simulink model "balance_and_leg_control"  (R2021b)
settings: Solver=ode4  StartTime=0.0  StopTime=12  FixedStep=1e-4  RelTol=1e-3
undefined symbols (not defined in the file): balance_controller_t, body, leg1, leg2, leg_controller_t, leg_fit_t, leg_t, param_t, sigbuilder_block, wheel, X, Y, Z
libraries: sm_lib x59, nesl_utility x15, slpidlib x2
(part 1 of 2)
settings Model: SimulationMode=accelerator  Creator=thinkpad  LastModifiedBy=thinkpad
settings OptimizationCC: DefaultUnderspecifiedDataType=single
settings ExplorerConfigSet: InternalSimMechanicsExplorerSettings="<ExplorerConfiguration><canonicalview>default</canonicalview><AnimationSetting><BasePlaybackSpeed>1.0</BasePlaybackSpeed><PlaybackSpeedFactor>1.0</PlaybackSpeedFactor></AnimationSetting><TilePanel><TileInfo><Tiles Columns=\"1\" Count=\"1\" Rows=\"1\"><Column Weight=\"1\"/><Row Weight=\"1\"/><Tile Height=\"1\" Width=\"1\" X=\"0\" Y=\"0\"/></Tiles></TileInfo><SceneInfo><SceneViewer><BGColor><R>0.815686285495758057</R><G>0.815686285495758057</G><B>0.815686285495758057</B></BGColor><Camera><DoPerspective>off</DoPerspective><Position><X>0.307352454887792503</X><Y>-1.00000000399907174</Y><Z>0.174322899702416489</Z></Position><Center><X>0.307352454887792503</X><Y>-3.99907176817926313e-09</Y><Z>0.174322899702416489</Z></Center><Up><X>0</X><Y>-0</Y><Z>1</Z></Up><ViewLimDist>1</ViewLimDist><YLim>0.280830658411598988</YLim><XLim>0.503375708473620787</XLim></Camera></SceneViewer></SceneInfo></TilePanel><MechEditorPanel><Cameras/><GfxPanelCameraMap/><VideoCreator><PlaybackSpeedRatio>1.0</PlaybackSpeedRatio><FrameRate>30</FrameRate><VideoFormat>Motion JPEG AVI</VideoFormat><FrameSize>[800 600]</FrameSize></VideoCreator></MechEditorPanel></ExplorerConfiguration>"

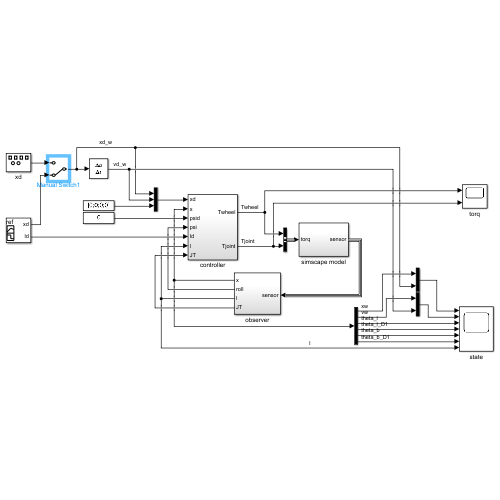
[thumbnail: Simulink's stored preview of the top-level diagram]
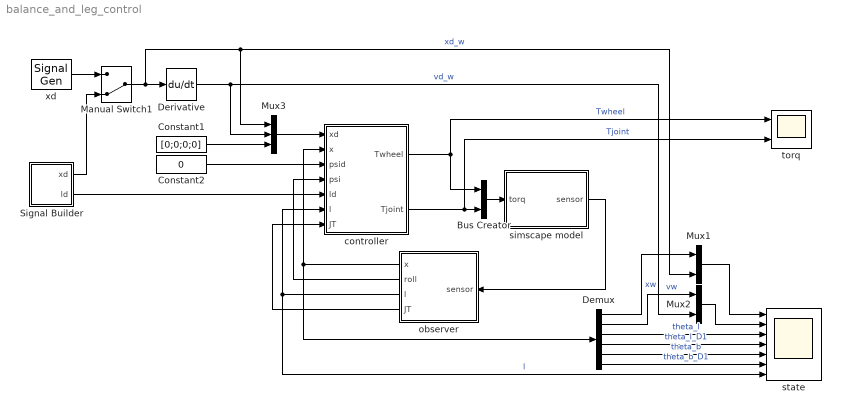
== system balance_and_leg_control ==
  Bus Creator : BusCreator  Inputs=2
  Constant1 : Constant  Value=[0;0;0;0]
  Constant2 : Constant  Value=0
  Demux : Demux  Outputs=6
  Derivative : Derivative
  Manual Switch1 : ManualSwitch  CurrentSetting=0
  Mux1 : Mux  Inputs=2
  Mux2 : Mux  Inputs=2
  Mux3 : Mux  Inputs=3
  Signal Builder : Subsystem  Tag=STV Subsys  LoadFcn=sigbuilder_block('load');  StartFcn=sigbuilder_block('start');  StopFcn=sigbuilder_block('stop');  ClipboardFcn=sigbuilder_block('clipboard');  mask(Sigbuilder block){tuvar=[0:10]}
      mask help: Simulink:masks:SigbuilderBlock_MD
      mask init:
      | if ~strcmp(get_param(bdroot(gcbh),'SimulationStatus'),'stopped') tuvar = sigbuilder_block('maskInit'); end
      settings: CopyFcn=sigbuilder_block('copy');  DeleteFcn=sigbuilder_block('delete');  ModelCloseFcn=sigbuilder_block('modelClose');  PreSaveFcn=sigbuilder_block('preSave');  PauseFcn=sigbuilder_block('pause');  ContinueFcn=sigbuilder_block('continue');  NameChangeFcn=sigbuilder_block('namechange');  OpenFcn=sigbuilder_block('open',[427.2 154.8 550.8 400.2 ]);  CloseFcn=sigbuilder_block('close');
      mask Display: plot(0, 0, 100, 100,[2, 2, 32, 32, 2], [68, 8, 8, 68, 68],[32, 2], [38, 38], [32, 19, 2],[53, 60, 44], [32, 17, 17, 2],[16, 16, 31, 31]);txt = getActiveGroup(gcbh);text(2, 100, txt,'verticalAlignment', 'top');
  controller : Subsystem
  observer : Subsystem
  simscape model : Subsystem
  state : Scope  NumInputPorts=7
  torq : Scope  NumInputPorts=2
  xd : SignalGenerator  WaveForm=square  Amplitude=0  Frequency=0.1
  wires:
  Manual Switch1/1 -> Mux1/2, Mux3/1, Derivative/1  "xd_w"
  Mux3/1 -> controller/1(xd)
  Constant1/1 -> Mux3/3
  Derivative/1 -> Mux3/2, Mux2/2  "vd_w"
  xd/1 -> Manual Switch1/1
  Signal Builder/1(xd) -> Manual Switch1/2
  controller/1(Twheel) -> torq/1, Bus Creator/1  "Twheel"
  controller/2(Tjoint) -> torq/2, Bus Creator/2  "Tjoint"
  Signal Builder/2(ld) -> controller/5(ld)
  Bus Creator/1 -> simscape model/1(torq)
  observer/4(JT) -> controller/7(JT)
  observer/3(l) -> state/7, controller/6(l)  "l"
  observer/2(roll) -> controller/4(psi)
  observer/1(x) -> controller/2(x), Demux/1
  Constant2/1 -> controller/3(psid)
  simscape model/1(sensor) -> observer/1(sensor)
  Demux/1 -> Mux1/1  "xw"
  Demux/2 -> Mux2/1  "vw"
  Mux1/1 -> state/1
  Mux2/1 -> state/2
  Demux/3 -> state/3  "theta_l"
  Demux/6 -> state/6  "theta_b_D1"
  Demux/5 -> state/5  "theta_b"
  Demux/4 -> state/4  "theta_l_D1"

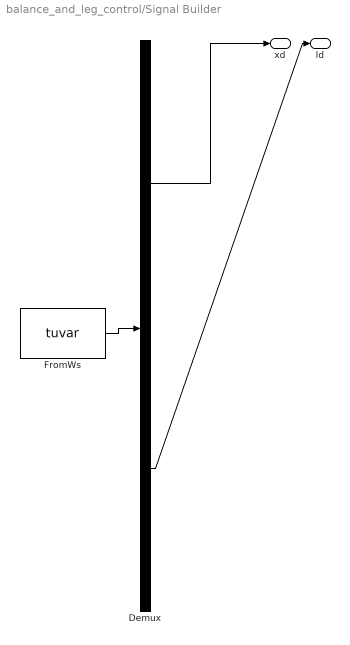
== system balance_and_leg_control/Signal Builder ==
  Demux : Demux  Tag=STV Demux  Outputs=2
      settings: DisplayOption=none
  FromWs : FromWorkspace  Tag=STV FromWs  VariableName=tuvar
      SigBuilderData=|
      | common.afterFinalStr = 'Extrapolate'
      | common.sampleTime = 0
      | dataSet.timeRange = [0 20]
      | dataSet.name = 'ref'
      | sbobj.Groups.Name = 'ref'
      | sbobj.Groups.Signals(1).Name = 'xd'
      | sbobj.Groups.Signals(1).XData = [0 1.5 2 4.5 7 10 20]
      | sbobj.Groups.Signals(1).YData = [0.1 -3.5 -3.5 4 4 0 0]
      | sbobj.Groups.Signals(2).Name = 'ld'
      | sbobj.Groups.Signals(2).XData = [0 20]
      | sbobj.Groups.Signals(2).YData = [0.24 0.24]
      | sbobj.Groups.TimeRange = [0 20]
  xd : Outport  Tag=STV Outport
  ld : Outport  Tag=STV Outport  Port=2
  wires:
  Demux/1 -> xd/1
  FromWs/1 -> Demux/1
  Demux/2 -> ld/1

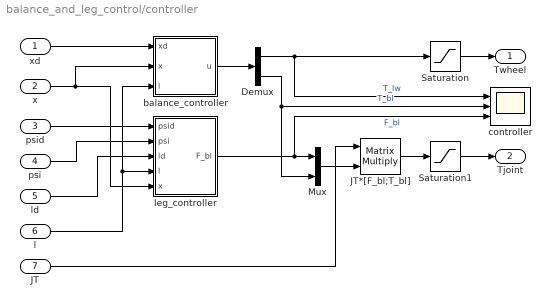
== system balance_and_leg_control/controller ==
  xd : Inport
  x : Inport  Port=2
  psid : Inport  Port=3
  psi : Inport  Port=4
  ld : Inport  Port=5
  l : Inport  Port=6
  JT : Inport  Port=7
  Demux : Demux  Outputs=2
  JT*[F_bl;T_bl] : Product  Multiplication=Matrix(*)
  Mux : Mux  Inputs=2
  Saturation : Saturate  UpperLimit=8  LowerLimit=-8
  Saturation1 : Saturate  UpperLimit=[70 70]  LowerLimit=-[70 70]
  balance_controller : Subsystem
  controller : Scope  NumInputPorts=3
  leg_controller : Subsystem
  Twheel : Outport
  Tjoint : Outport  Port=2
  wires:
  xd/1 -> balance_controller/1(xd)
  x/1 -> leg_controller/5(x), balance_controller/2(x)
  balance_controller/1(u) -> Demux/1
  Demux/1 -> Saturation/1, controller/1  "T_lw"
  leg_controller/1(F_bl) -> controller/3, Mux/1  "F_bl"
  Demux/2 -> controller/2, Mux/2  "T_bl"
  l/1 -> balance_controller/3(l), leg_controller/4(l)
  psid/1 -> leg_controller/1(psid)
  psi/1 -> leg_controller/2(psi)
  ld/1 -> leg_controller/3(ld)
  Mux/1 -> JT*[F_bl;T_bl]/2
  JT*[F_bl;T_bl]/1 -> Saturation1/1
  JT/1 -> JT*[F_bl;T_bl]/1
  Saturation/1 -> Twheel/1
  Saturation1/1 -> Tjoint/1

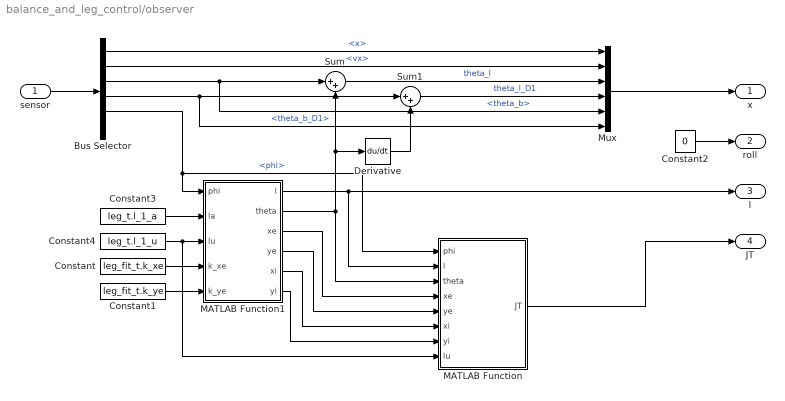
== system balance_and_leg_control/observer ==
  sensor : Inport
  Bus Selector : BusSelector  OutputSignals=x,vx,theta_b,theta_b_D1,phi,phi_D1
  Constant : Constant  Value=leg_fit_t.k_xe
  Constant1 : Constant  Value=leg_fit_t.k_ye
  Constant2 : Constant  Value=0
  Constant3 : Constant  Value=leg_t.l_1_a
  Constant4 : Constant  Value=leg_t.l_1_u
  Derivative : Derivative
  MATLAB Function : MATLAB Function  TreatAsAtomicUnit=on
  MATLAB Function1 : MATLAB Function  TreatAsAtomicUnit=on
  Mux : Mux  Inputs=6
  Sum : Sum  Inputs=|++
  Sum1 : Sum  Inputs=|++
  x : Outport
  roll : Outport  Port=2
  l : Outport  Port=3
  JT : Outport  Port=4
  wires:
  MATLAB Function1/1(l) -> l/1, MATLAB Function/2(l)
  MATLAB Function1/2(theta) -> Sum/2, Derivative/1, MATLAB Function/3(theta)
  MATLAB Function/1(JT) -> JT/1
  sensor/1 -> Bus Selector/1
  Mux/1 -> x/1
  Bus Selector/1 -> Mux/1  "<x>"
  Bus Selector/2 -> Mux/2  "<vx>"
  Constant2/1 -> roll/1
  Bus Selector/3 -> Sum/1, Mux/5  "<theta_b>"
  Bus Selector/4 -> Sum1/1, Mux/6  "<theta_b_D1>"
  Bus Selector/5 -> MATLAB Function1/1(phi), MATLAB Function/1(phi)  "<phi>"
  Constant/1 -> MATLAB Function1/4(k_xe)
  Constant1/1 -> MATLAB Function1/5(k_ye)
  Sum/1 -> Mux/3  "theta_l"
  Sum1/1 -> Mux/4  "theta_l_D1"
  Derivative/1 -> Sum1/2
  Constant3/1 -> MATLAB Function1/2(la)
  Constant4/1 -> MATLAB Function1/3(lu), MATLAB Function/8(lu)
  MATLAB Function1/3(xe) -> MATLAB Function/4(xe)
  MATLAB Function1/4(ye) -> MATLAB Function/5(ye)
  MATLAB Function1/5(xi) -> MATLAB Function/6(xi)
  MATLAB Function1/6(yi) -> MATLAB Function/7(yi)

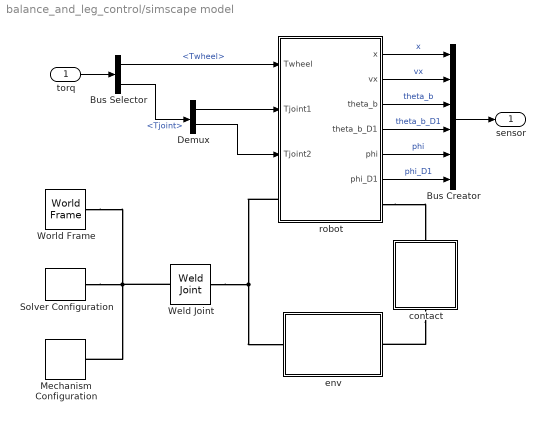
== system balance_and_leg_control/simscape model ==
  torq : Inport
  Bus Creator : BusCreator  Inputs=6
  Bus Selector : BusSelector  OutputSignals=Twheel,Tjoint
  Demux : Demux  Outputs=2
  Mechanism Configuration : sm_lib/Utilities/Mechanism Configuration  UniformGravity=Constant  GravityVector=[0 0 -9.81]  GravityUnits=m/s^2  LinearizationDelta=0.001  JointModeTransitionNonlinearIterations=2
  Solver Configuration : nesl_utility/Solver Configuration  PhysicalDomain=network_engine_domain  SubClassName=solver  LeftPortType=input  RightPortType=generic  Tones=[]  Harmonics=[]  SimulateNoise=off  Profile=off  UseLocalSampling=off  EnableSwitchedLinearOptims=on  FrequencyDomain=off  UseCCode=off  RelTol=0.001  AbsTol=1e-06  MinStep=1e-09  ToWorkspace=off  RevertToSquareIcSolve=off  NumHomotopyIterations=100  PhasorMode=off  PhasorModeNumHarmonics=1  DoDC=off  ResidualTolerance=1e-09  UseLocalSolver=off  LocalSolverChoice=NE_BACKWARD_EULER_ADVANCER  LocalSolverSampleTime=0.001  DoFixedCost=off  MaxNonlinIter=3  MaxModeIter=2  ComputeImpulses=off  ImpulseIterations=2  LinearAlgebra=Sparse  EquationFormulation=NE_TIME_EF  DelaysMemoryBudget=1024  AutomaticFiltering=on  FilteringTimeConstant=0.001  PartitionStorageMethod=AS_NEEDED  PartitionMemoryBudget=1024  PartitionMethod=FAST
      settings: SourceProductBaseCode=PW,SS
  Weld Joint : sm_lib/Joints/Weld Joint  JointMode=Normal  SenseConstraintForce=off  SenseConstraintForceX=off  SenseConstraintForceY=off  SenseConstraintForceZ=off  SenseConstraintTorque=off  SenseConstraintTorqueX=off  SenseConstraintTorqueY=off  SenseConstraintTorqueZ=off  SenseTotalForce=off  SenseTotalForceX=off  SenseTotalForceY=off  SenseTotalForceZ=off  SenseTotalTorque=off  SenseTotalTorqueX=off  SenseTotalTorqueY=off  SenseTotalTorqueZ=off  CompositeWrenchDir=FollowerOnBase  CompositeWrenchFrame=BaseFrame
  World Frame : sm_lib/Frames and Transforms/World Frame
  contact : Subsystem
      settings: PortSchema="{\"entries\":[{\"content\":{\"sides\":[{\"content\":{\"connectorIds\":[]},\"type\":\"ConnectorPlacement.EquallySpacedRectSide\",\"uuid\":\"948d884d-a2bb-4982-bec2-8891ab05edb1\"},{\"content\":{\"connectorIds\":[],\"side\":\"RIGHT\"},\"type\":\"ConnectorPlacement.EquallySpacedRectSide\",\"uuid\":\"1ab48329-b8c1-41fb-bc52-c8a32a07fc10\"},{\"content\":{\"connectorIds\":[\"LConn1\"],\"side\":\"TOP\"},\"type\":\"ConnectorPlacement.EquallySpacedRectSide\",\"uuid\":\"2430d379-17bc-45a7-9277-8300fd306697\"},{\"content\":{\"connectorIds\":[\"RConn1\"],\"side\":\"BOTTOM\"},\"type\":\"ConnectorPlacement.EquallySpacedRectSide\",\"uuid\":\"c2c22df6-47ef-4364-9ed6-2fe5d2ebd561\"}]},\"type\":\"ConnectorPlacement.EquallySpacedConnector\",\"uuid\":\"bd96c317-3050-474a-affa-ffce42783eb1\"}],\"packageUris\":[\"http://schema.mathworks.com/mf0/Connector/R2020b\"],\"version\":\"1.0\"}"
  env : Subsystem
  robot : Subsystem
  sensor : Outport
  wires:
  torq/1 -> Bus Selector/1
  Bus Selector/2 -> Demux/1  "<Tjoint>"
  Demux/1 -> robot/2(Tjoint1)
  Demux/2 -> robot/3(Tjoint2)
  Bus Creator/1 -> sensor/1
  robot/1(x) -> Bus Creator/1  "x"
  robot/2(vx) -> Bus Creator/2  "vx"
  robot/3(theta_b) -> Bus Creator/3  "theta_b"
  robot/4(theta_b_D1) -> Bus Creator/4  "theta_b_D1"
  robot/5(phi) -> Bus Creator/5  "phi"
  robot/6(phi_D1) -> Bus Creator/6  "phi_D1"
  Bus Selector/1 -> robot/1(Twheel)  "<Twheel>"
  connections:
  World Frame/RConn1 -- Weld Joint/LConn1 -- Mechanism Configuration/RConn1 -- Solver Configuration/RConn1
  contact/RConn1 -- env/RConn1
  Weld Joint/RConn1 -- env/LConn1 -- robot/LConn1
  robot/RConn1 -- contact/LConn1

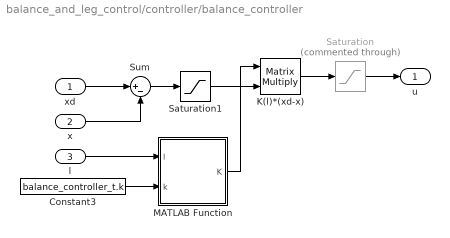
== system balance_and_leg_control/controller/balance_controller ==
  xd : Inport
  x : Inport  Port=2
  l : Inport  Port=3
  Constant3 : Constant  Value=balance_controller_t.k
  K(l)*(xd-x) : Product  Multiplication=Matrix(*)
  MATLAB Function : MATLAB Function  TreatAsAtomicUnit=on
  Saturation : Saturate  Commented=through  UpperLimit=1  LowerLimit=-1
  Saturation1 : Saturate  UpperLimit=[0.5,3,inf,inf,inf,inf]  LowerLimit=-[0.5,3,inf,inf,inf,inf]
  Sum : Sum  Inputs=|+-
  u : Outport
  wires:
  Saturation/1 -> u/1
  Saturation1/1 -> K(l)*(xd-x)/2
  MATLAB Function/1(K) -> K(l)*(xd-x)/1
  l/1 -> MATLAB Function/1(l)
  x/1 -> Sum/2
  xd/1 -> Sum/1
  Sum/1 -> Saturation1/1
  K(l)*(xd-x)/1 -> Saturation/1
  Constant3/1 -> MATLAB Function/2(k)

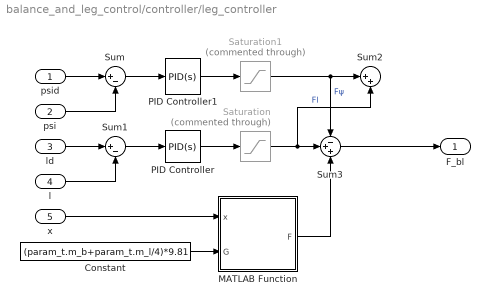
== system balance_and_leg_control/controller/leg_controller ==
  psid : Inport
  psi : Inport  Port=2
  ld : Inport  Port=3
  l : Inport  Port=4
  x : Inport  Port=5
  Constant : Constant  Value=(param_t.m_b+param_t.m_l/4)*9.81
  MATLAB Function : MATLAB Function  TreatAsAtomicUnit=on
  PID Controller : slpidlib/PID Controller  Controller=PID  Form=Parallel  TimeDomain=Continuous-time  UseExternalTs=off  SampleTime=-1  IntegratorMethod=Forward Euler  FilterMethod=Forward Euler  ControllerParametersSource=internal  P=leg_controller_t.l.kp  I=leg_controller_t.l.ki  D=leg_controller_t.l.kd  UseFilter=on  N=100  TunerSelectOption=Transfer Function Based (PID Tuner App)  InitialConditionSource=internal  InitialConditionForIntegrator=0  InitialConditionForFilter=0  DifferentiatorICPrevScaledInput=0  ExternalReset=none  TrackingMode=off  Kt=1  LimitOutput=off  SatLimitsSource=internal  UpperSaturationLimit=inf  LowerSaturationLimit=-inf  LinearizeAsGain=on  AntiWindupMode=none  Kb=1  POutMin=[]  POutMax=[]  IOutMin=[]  IOutMax=[]  DOutMin=[]  DOutMax=[]  NOutMin=[]  NOutMax=[]  SumOutMin=[]  SumOutMax=[]  SaturationOutMin=[]  SaturationOutMax=[]  PParamMin=[]  PParamMax=[]  IParamMin=[]  IParamMax=[]  DParamMin=[]  DParamMax=[]  NParamMin=[]  NParamMax=[]  KbParamMin=[]  KbParamMax=[]  KtParamMin=[]  KtParamMax=[]  KbOutMin=[]  KbOutMax=[]  KtOutMin=[]  KtOutMax=[]  IntegratorOutMin=[]  IntegratorOutMax=[]  FilterOutMin=[]  FilterOutMax=[]  SumI1OutMin=[]  SumI1OutMax=[]  SumI2OutMin=[]  SumI2OutMax=[]  SumI3OutMin=[]  SumI3OutMax=[]  SumI4OutMin=[]  SumI4OutMax=[]  SumDOutMin=[]  SumDOutMax=[]  DifferentiatorOutMin=[]  DifferentiatorOutMax=[]  FilterDiffOutCoefMin=[]  FilterDiffOutCoefMax=[]  ReciprocalOutMin=[]  ReciprocalOutMax=[]  SumDenOutMin=[]  SumDenOutMax=[]  SumNumOutMin=[]  SumNumOutMax=[]  DivideOutMin=[]  DivideOutMax=[]  UdiffTsProdOutMin=[]  UdiffTsProdOutMax=[]  NTsProdOutMin=[]  NTsProdOutMax=[]  UintegralTsProdOutMin=[]  UintegralTsProdOutMax=[]  UngainTsProdOutMin=[]  UngainTsProdOutMax=[]  IntegratorContinuousStateAttributes=''  IntegratorStateMustResolveToSignalObject=off  IntegratorRTWStateStorageClass=Auto  FilterContinuousStateAttributes=''  FilterStateMustResolveToSignalObject=off  FilterRTWStateStorageClass=Auto  ParallelPVariant=InternalParameters  IdealPVariant=Disabled  IVariant=InternalParameters  DVariant=InternalParameters  IntegratorVariant=Continuous  SatVariant=Disabled  AWVariant=Passthrough  PCopyVariant=Disabled  TRVariant=Disabled  FdbkBlocksVariant=Forward  IdealPFdbkVariant=Disabled  SatFdbkVariant=Disabled  DerivativeFilterVariant=ContFilter  NVariant=InternalParameters  NCopyVariant=Disabled  FilterICVariant=InternalICsFilter  IntegratorICVariant=InternalICs  ExternalResetVariant=Disabled  TRSumVariant=Passthrough  SumFdbkVariant=Disabled  SumVariant=Sum_PID  TsampFilterVariant=InternalTs  TsampNgainVariant=Passthrough  TsampIntegralVariant=Passthrough  ExternalSaturationOutDataTypeStr=Inherit: Same as second input
  PID Controller1 : slpidlib/PID Controller  Controller=PID  Form=Parallel  TimeDomain=Continuous-time  UseExternalTs=off  SampleTime=-1  IntegratorMethod=Forward Euler  FilterMethod=Forward Euler  ControllerParametersSource=internal  P=leg_controller_t.psi.kp  I=leg_controller_t.psi.ki  D=leg_controller_t.psi.kd  UseFilter=on  N=100  TunerSelectOption=Transfer Function Based (PID Tuner App)  InitialConditionSource=internal  InitialConditionForIntegrator=0  InitialConditionForFilter=0  DifferentiatorICPrevScaledInput=0  ExternalReset=none  TrackingMode=off  Kt=1  LimitOutput=off  SatLimitsSource=internal  UpperSaturationLimit=inf  LowerSaturationLimit=-inf  LinearizeAsGain=on  AntiWindupMode=none  Kb=1  POutMin=[]  POutMax=[]  IOutMin=[]  IOutMax=[]  DOutMin=[]  DOutMax=[]  NOutMin=[]  NOutMax=[]  SumOutMin=[]  SumOutMax=[]  SaturationOutMin=[]  SaturationOutMax=[]  PParamMin=[]  PParamMax=[]  IParamMin=[]  IParamMax=[]  DParamMin=[]  DParamMax=[]  NParamMin=[]  NParamMax=[]  KbParamMin=[]  KbParamMax=[]  KtParamMin=[]  KtParamMax=[]  KbOutMin=[]  KbOutMax=[]  KtOutMin=[]  KtOutMax=[]  IntegratorOutMin=[]  IntegratorOutMax=[]  FilterOutMin=[]  FilterOutMax=[]  SumI1OutMin=[]  SumI1OutMax=[]  SumI2OutMin=[]  SumI2OutMax=[]  SumI3OutMin=[]  SumI3OutMax=[]  SumI4OutMin=[]  SumI4OutMax=[]  SumDOutMin=[]  SumDOutMax=[]  DifferentiatorOutMin=[]  DifferentiatorOutMax=[]  FilterDiffOutCoefMin=[]  FilterDiffOutCoefMax=[]  ReciprocalOutMin=[]  ReciprocalOutMax=[]  SumDenOutMin=[]  SumDenOutMax=[]  SumNumOutMin=[]  SumNumOutMax=[]  DivideOutMin=[]  DivideOutMax=[]  UdiffTsProdOutMin=[]  UdiffTsProdOutMax=[]  NTsProdOutMin=[]  NTsProdOutMax=[]  UintegralTsProdOutMin=[]  UintegralTsProdOutMax=[]  UngainTsProdOutMin=[]  UngainTsProdOutMax=[]  IntegratorContinuousStateAttributes=''  IntegratorStateMustResolveToSignalObject=off  IntegratorRTWStateStorageClass=Auto  FilterContinuousStateAttributes=''  FilterStateMustResolveToSignalObject=off  FilterRTWStateStorageClass=Auto  ParallelPVariant=InternalParameters  IdealPVariant=Disabled  IVariant=InternalParameters  DVariant=InternalParameters  IntegratorVariant=Continuous  SatVariant=Disabled  AWVariant=Passthrough  PCopyVariant=Disabled  TRVariant=Disabled  FdbkBlocksVariant=Forward  IdealPFdbkVariant=Disabled  SatFdbkVariant=Disabled  DerivativeFilterVariant=ContFilter  NVariant=InternalParameters  NCopyVariant=Disabled  FilterICVariant=InternalICsFilter  IntegratorICVariant=InternalICs  ExternalResetVariant=Disabled  TRSumVariant=Passthrough  SumFdbkVariant=Disabled  SumVariant=Sum_PID  TsampFilterVariant=InternalTs  TsampNgainVariant=Passthrough  TsampIntegralVariant=Passthrough  ExternalSaturationOutDataTypeStr=Inherit: Same as second input
  Saturation : Saturate  Commented=through  UpperLimit=30  LowerLimit=-30
  Saturation1 : Saturate  Commented=through  UpperLimit=30  LowerLimit=-30
  Sum : Sum  Inputs=|+-
  Sum1 : Sum  Inputs=|+-
  Sum2 : Sum  Inputs=|++
  Sum3 : Sum  Inputs=-++
  F_bl : Outport
  wires:
  psi/1 -> Sum/2
  l/1 -> Sum1/2
  ld/1 -> Sum1/1
  psid/1 -> Sum/1
  Sum1/1 -> PID Controller/1
  Sum/1 -> PID Controller1/1
  PID Controller1/1 -> Saturation1/1
  PID Controller/1 -> Saturation/1
  Saturation1/1 -> Sum3/1, Sum2/1  "Fψ"
  Saturation/1 -> Sum2/2, Sum3/2  "Fl"
  Sum3/1 -> F_bl/1
  Constant/1 -> MATLAB Function/2(G)
  x/1 -> MATLAB Function/1(x)
  MATLAB Function/1(F) -> Sum3/3

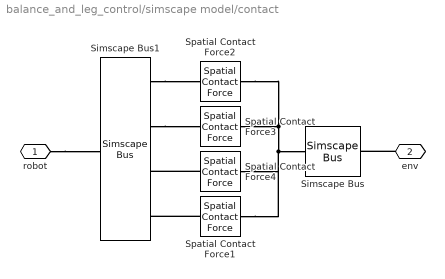
== system balance_and_leg_control/simscape model/contact ==
  Simscape Bus : SimscapeBus  HierarchyStrings=ground
  Simscape Bus1 : SimscapeBus  HierarchyStrings=body;leg1;leg2;wheel
  Spatial Contact Force1 : sm_lib/Forces and Torques/Spatial Contact Force  CoefficientOfDynamicFriction=0.3  CoefficientOfStaticFriction=0.5  SenseContactBaseRotation=off  SenseContactBaseTranslation=off  NormalDamping=1e5  NormalDampingUnits=N/(m/s)  SenseContactFollowerRotation=off  SenseContactFollowerTranslation=off  SenseContactSignal=off  NormalStiffness=1e6  NormalStiffnessUnits=N/m  FrictionalCriticalVelocity=1e-3  FrictionalCriticalVelocityUnits=m/s  ZeroCrossDetectContactStartAndEnd=off  FrictionType=SmoothStickSlip  SenseFrictionalForceMagnitude=off  SenseNormalForceMagnitude=off  NormalForceType=SmoothSpringDamper  SenseNormalVelocity=off  SenseSeparationDistance=off  SenseTangentialVelocity=off  SenseTangentialVelocityMagnitude=off  NormalTransitionRegionWidth=1e-4  NormalTransitionRegionWidthUnits=m
  Spatial Contact Force2 : sm_lib/Forces and Torques/Spatial Contact Force  CoefficientOfDynamicFriction=0.3  CoefficientOfStaticFriction=0  SenseContactBaseRotation=off  SenseContactBaseTranslation=off  NormalDamping=1e5  NormalDampingUnits=N/(m/s)  SenseContactFollowerRotation=off  SenseContactFollowerTranslation=off  SenseContactSignal=off  NormalStiffness=1e6  NormalStiffnessUnits=N/m  FrictionalCriticalVelocity=1e-3  FrictionalCriticalVelocityUnits=m/s  ZeroCrossDetectContactStartAndEnd=off  FrictionType=SmoothStickSlip  SenseFrictionalForceMagnitude=off  SenseNormalForceMagnitude=off  NormalForceType=SmoothSpringDamper  SenseNormalVelocity=off  SenseSeparationDistance=off  SenseTangentialVelocity=off  SenseTangentialVelocityMagnitude=off  NormalTransitionRegionWidth=1e-4  NormalTransitionRegionWidthUnits=m
  Spatial Contact Force3 : sm_lib/Forces and Torques/Spatial Contact Force  CoefficientOfDynamicFriction=0.3  CoefficientOfStaticFriction=0  SenseContactBaseRotation=off  SenseContactBaseTranslation=off  NormalDamping=1e5  NormalDampingUnits=N/(m/s)  SenseContactFollowerRotation=off  SenseContactFollowerTranslation=off  SenseContactSignal=off  NormalStiffness=1e6  NormalStiffnessUnits=N/m  FrictionalCriticalVelocity=1e-3  FrictionalCriticalVelocityUnits=m/s  ZeroCrossDetectContactStartAndEnd=off  FrictionType=SmoothStickSlip  SenseFrictionalForceMagnitude=off  SenseNormalForceMagnitude=off  NormalForceType=SmoothSpringDamper  SenseNormalVelocity=off  SenseSeparationDistance=off  SenseTangentialVelocity=off  SenseTangentialVelocityMagnitude=off  NormalTransitionRegionWidth=1e-4  NormalTransitionRegionWidthUnits=m
  Spatial Contact Force4 : sm_lib/Forces and Torques/Spatial Contact Force  CoefficientOfDynamicFriction=0.3  CoefficientOfStaticFriction=0  SenseContactBaseRotation=off  SenseContactBaseTranslation=off  NormalDamping=1e5  NormalDampingUnits=N/(m/s)  SenseContactFollowerRotation=off  SenseContactFollowerTranslation=off  SenseContactSignal=off  NormalStiffness=1e6  NormalStiffnessUnits=N/m  FrictionalCriticalVelocity=1e-3  FrictionalCriticalVelocityUnits=m/s  ZeroCrossDetectContactStartAndEnd=off  FrictionType=SmoothStickSlip  SenseFrictionalForceMagnitude=off  SenseNormalForceMagnitude=off  NormalForceType=SmoothSpringDamper  SenseNormalVelocity=off  SenseSeparationDistance=off  SenseTangentialVelocity=off  SenseTangentialVelocityMagnitude=off  NormalTransitionRegionWidth=1e-4  NormalTransitionRegionWidthUnits=m
  robot : PMIOPort  Side=Left
  env : PMIOPort  Port=2  Side=Right
  connections:
  Spatial Contact Force4/LConn1 -- Simscape Bus1/LConn3
  env/RConn1 -- Simscape Bus/RConn1
  robot/RConn1 -- Simscape Bus1/RConn1
  Simscape Bus1/LConn1 -- Spatial Contact Force2/LConn1
  Spatial Contact Force2/RConn1 -- Spatial Contact Force1/RConn1 -- Spatial Contact Force4/RConn1 -- Simscape Bus/LConn1 -- Spatial Contact Force3/RConn1
  Spatial Contact Force1/LConn1 -- Simscape Bus1/LConn4
  Simscape Bus1/LConn2 -- Spatial Contact Force3/LConn1

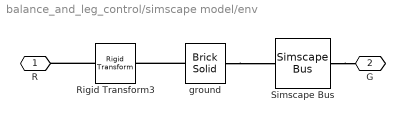
== system balance_and_leg_control/simscape model/env ==
  Rigid Transform3 : sm_lib/Frames and Transforms/Rigid Transform  TranslationMethod=StandardAxis  TranslationStandardOffset=-0.05  TranslationLengthUnit=m  TranslationStandardAxis=+Z  TranslationCartesianOffset=[0 0 0]  TranslationROffset=0  TranslationROffsetUnits=m  TranslationZOffset=0  TranslationZOffsetUnits=m  TranslationThetaOffset=0  TranslationThetaOffsetUnits=deg  RotationMethod=None  RotationAngleUnits=deg  RotationStandardAxis=+X  RotationAngle=90  RotationArbitraryAxis=[0 0 1]  FollAlignAxisA=+X  BaseAlignAxisA=+Y  FollAlignAxisB=+Y  BaseAlignAxisB=+Z  RotationSequenceAxes=FollowerAxes  RotationSequence=XYX  RotationSequenceAngles=[0 0 0]  RotationSequenceAnglesUnits=deg  RotationMatrix=[1 0 0; 0 1 0; 0 0 1]
  Simscape Bus : SimscapeBus  HierarchyStrings=ground
  ground : sm_lib/Body Elements/Brick Solid  GraphicAmbientColor=[0.15 0.15 0.15 1.0]  BasedOnType=Density  BrickDimensions=[10 1 0.1]  BrickDimensionUnits=m  CenterOfMass=[0 0 0]  CenterOfMassUnits=m  GraphicDiffuseColor=[0.9 0.9 0.9]  Density=1000  DensityUnits=kg/m^3  DoExposeReferenceFrame=on  GraphicEmissiveColor=[0.0 0.0 0.0 1.0]  ExportEntireGeometry=on  SerializedFrames=<Frames/>  MarkerShape=Sphere  MarkerSize=10  GraphicType=FromGeometry  InertiaType=CalculateFromGeometry  Mass=1  MassUnits=kg  MomentsOfInertia=[1 1 1]  MomentsOfInertiaUnits=kg*m^2  GraphicOpacity=1.0  ProductsOfInertia=[0 0 0]  ProductsOfInertiaUnits=kg*m^2  GraphicShininess=75  GraphicSpecularColor=[0.5 0.5 0.5 1.0]  GraphicVisPropType=SimpleVisualProperties
  R : PMIOPort  Side=Left
  G : PMIOPort  Port=2  Side=Right
  connections:
  Simscape Bus/RConn1 -- G/RConn1
  ground/RConn1 -- Rigid Transform3/RConn1
  ground/LConn1 -- Simscape Bus/LConn1
  Rigid Transform3/LConn1 -- R/RConn1
